simulink model "testing"  (R2025b)
settings: Solver=VariableStepAuto  StartTime=0.0  StopTime=50  RelTol=1e-3
values from neighbouring files (symbols this model uses):
  Area = 2*L*Width    (= 0.072)    [quad_params.m]
  end_h = 0.03    [quad_params.m]
  g = 9.81    [quad_params.m]
  h = [0 ... (first row only)    [Madgwick.m]    (also in quad_params.m = 0.2; umich_learning.m = x(:,1))
  h0 = Ts    (= 0.001)    [quad_params.m]
  inertia_mx = [Ixx; Iyy; Izz;]    [quad_params.m]
  init_h = 0.03    [quad_params.m]
  K_alloc = Alloc \ diag([W, 1, 1, 1])    [quad_params.m]
  r0_angle = 1000    [quad_params.m]
  r0_position = 1    [quad_params.m]
  rho_air = 1.225    [quad_params.m]
  rho_water = 1000    [quad_params.m]
  Trot = 0.01    [quad_params.m]
  Ts = 0.001    [get_noise.m]    (also in quad_params.m; test.m = 0.002)
  W = 0.7 + 4*m_prop    (= 0.74)    [quad_params.m]
undefined symbols (not defined in the file or in its folder): Alloc_2, b0, b0_pitch, b0_roll, b0_x, b0_y, b0_yaw, b0_z, beta1_pitch, beta1_roll, beta1_x, beta1_y, beta1_yaw, beta1_z, beta2_pitch, beta2_roll, beta2_x, beta2_y, beta2_yaw, beta2_z, beta3_pitch, beta3_roll, beta3_x, beta3_y, beta3_yaw, beta3_z, m, wc, wc_pitch, wc_roll, wc_x, wc_y, wc_yaw, wc_z, wo
libraries: simulink x3, shareduavrstlib x2, SignalEditorBlockLib x2, aerolibwind2 x1
(part 1 of 2)
settings Model: Creator=David  LastModifiedBy=David

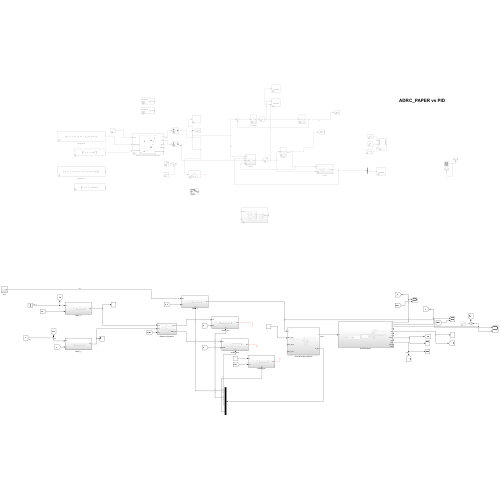
[thumbnail: Simulink's stored preview of the top-level diagram]
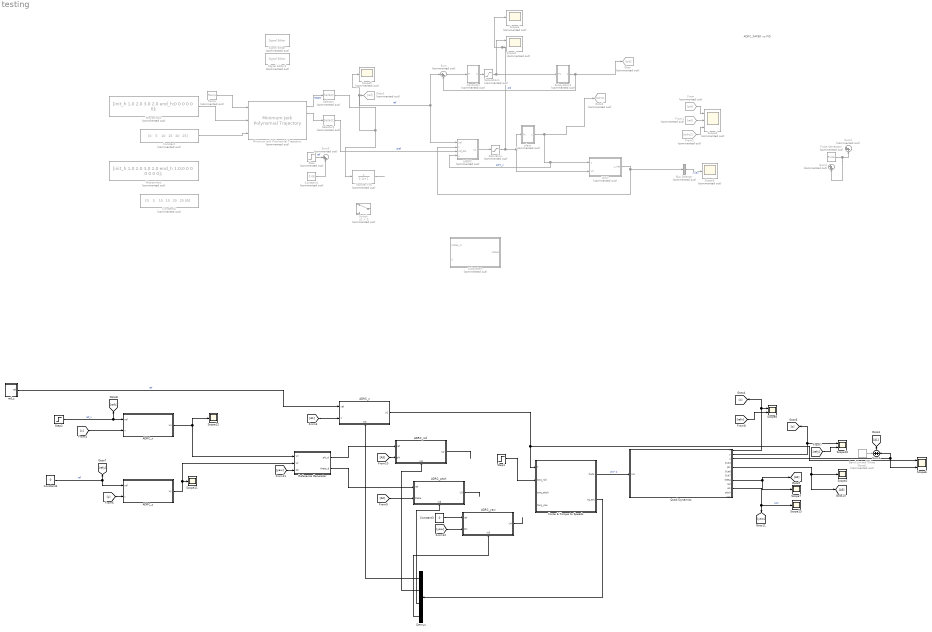
== system testing ==
  note: ADRC_PAPER vs PID
  ADRC_pitch : Subsystem
      settings: PortSchema="{\"entries\":[{\"content\":{\"sides\":[{\"content\":{\"connectorIds\":[\"In1\",\"In2\"]},\"type\":\"ConnectorPlacement.EquallySpacedRectSide\",\"uuid\":\"6cc80560-d5fb-4d70-bab2-c51ed037dc75\"},{\"content\":{\"connectorIds\":[\"Out1\"],\"side\":\"RIGHT\"},\"type\":\"ConnectorPlacement.EquallySpacedRectSide\",\"uuid\":\"11bda7cd-3ac7-47c0-848b-d0ab204a3c3d\"},{\"content\":{\"side\":\"TOP\"},\"type\":\"ConnectorPlacement.EquallySpacedRectSide\",\"uuid\":\"2a4fd4ae-6a0e-48eb-9f11-b11d2041070f\"},{\"content\":{\"connectorIds\":[\"In3\"],\"side\":\"BOTTOM\"},\"type\":\"ConnectorPlacement.EquallySpacedRectSide\",\"uuid\":\"f4a2dede-c3a4-45a0-96a3-5f68fdbf4ab0\"}]},\"type\":\"ConnectorPlacement.EquallySpacedConnector\",\"uuid\":\"bf44a222-f2d1-4d7f-8b8f-a2aef4aa21c8\"}],\"packageUris\":[\"http://schema.mathworks.com/mf0/Connector/R2020b\"],\"version\":\"1.0\"}"
  ADRC_roll : Subsystem
      settings: PortSchema="{\"entries\":[{\"content\":{\"sides\":[{\"content\":{\"connectorIds\":[\"In1\",\"In2\"]},\"type\":\"ConnectorPlacement.EquallySpacedRectSide\",\"uuid\":\"6cc80560-d5fb-4d70-bab2-c51ed037dc75\"},{\"content\":{\"connectorIds\":[\"Out1\"],\"side\":\"RIGHT\"},\"type\":\"ConnectorPlacement.EquallySpacedRectSide\",\"uuid\":\"11bda7cd-3ac7-47c0-848b-d0ab204a3c3d\"},{\"content\":{\"side\":\"TOP\"},\"type\":\"ConnectorPlacement.EquallySpacedRectSide\",\"uuid\":\"2a4fd4ae-6a0e-48eb-9f11-b11d2041070f\"},{\"content\":{\"connectorIds\":[\"In3\"],\"side\":\"BOTTOM\"},\"type\":\"ConnectorPlacement.EquallySpacedRectSide\",\"uuid\":\"852e14b7-d2e0-4511-9e4e-b55cc1d4afdd\"}]},\"type\":\"ConnectorPlacement.EquallySpacedConnector\",\"uuid\":\"bf44a222-f2d1-4d7f-8b8f-a2aef4aa21c8\"}],\"packageUris\":[\"http://schema.mathworks.com/mf0/Connector/R2020b\"],\"version\":\"1.0\"}"
  ADRC_x : Subsystem
  ADRC_y : Subsystem
  ADRC_yaw : Subsystem
      settings: PortSchema="{\"entries\":[{\"content\":{\"sides\":[{\"content\":{\"connectorIds\":[\"In1\",\"In2\"]},\"type\":\"ConnectorPlacement.EquallySpacedRectSide\",\"uuid\":\"6cc80560-d5fb-4d70-bab2-c51ed037dc75\"},{\"content\":{\"connectorIds\":[\"Out1\"],\"side\":\"RIGHT\"},\"type\":\"ConnectorPlacement.EquallySpacedRectSide\",\"uuid\":\"11bda7cd-3ac7-47c0-848b-d0ab204a3c3d\"},{\"content\":{\"side\":\"TOP\"},\"type\":\"ConnectorPlacement.EquallySpacedRectSide\",\"uuid\":\"2a4fd4ae-6a0e-48eb-9f11-b11d2041070f\"},{\"content\":{\"connectorIds\":[\"In3\"],\"side\":\"BOTTOM\"},\"type\":\"ConnectorPlacement.EquallySpacedRectSide\",\"uuid\":\"76ba5801-5866-4633-be25-22afc3afb05e\"}]},\"type\":\"ConnectorPlacement.EquallySpacedConnector\",\"uuid\":\"bf44a222-f2d1-4d7f-8b8f-a2aef4aa21c8\"}],\"packageUris\":[\"http://schema.mathworks.com/mf0/Connector/R2020b\"],\"version\":\"1.0\"}"
  ADRC_z : Subsystem
      settings: PortSchema="{\"entries\":[{\"content\":{\"sides\":[{\"content\":{\"connectorIds\":[\"In1\",\"In2\"]},\"type\":\"ConnectorPlacement.EquallySpacedRectSide\",\"uuid\":\"6cc80560-d5fb-4d70-bab2-c51ed037dc75\"},{\"content\":{\"connectorIds\":[\"Out1\"],\"side\":\"RIGHT\"},\"type\":\"ConnectorPlacement.EquallySpacedRectSide\",\"uuid\":\"11bda7cd-3ac7-47c0-848b-d0ab204a3c3d\"},{\"content\":{\"side\":\"TOP\"},\"type\":\"ConnectorPlacement.EquallySpacedRectSide\",\"uuid\":\"2a4fd4ae-6a0e-48eb-9f11-b11d2041070f\"},{\"content\":{\"connectorIds\":[\"In3\"],\"side\":\"BOTTOM\"},\"type\":\"ConnectorPlacement.EquallySpacedRectSide\",\"uuid\":\"eaf2a28a-e13e-4347-87b8-9ecab679d798\"}]},\"type\":\"ConnectorPlacement.EquallySpacedConnector\",\"uuid\":\"bf44a222-f2d1-4d7f-8b8f-a2aef4aa21c8\"}],\"packageUris\":[\"http://schema.mathworks.com/mf0/Connector/R2020b\"],\"version\":\"1.0\"}"
  Band-Limited White Noise1 : simulink/Sources/Band-Limited White Noise  Commented=on  Cov=[2.5*10^-9]  Ts=Ts  seed=[23341]
  Bus Selector : BusSelector  Commented=on  OutputSignals=x3
  Constant : Constant  Commented=on  Value="[0    5    10   15   20   25]"
  Constant1 : Constant  Commented=on  Value=0.06
  Constant2 : Constant  Commented=on  Value="[0    5    10   15   20   25 30]"
  Constant3 : Constant  Value=0
  Constant4 : Constant  Value=0
  Controller : Subsystem  Commented=on
  Demux : Demux
  Force & Torque to Speeds : Subsystem
  From : From  Commented=on  GotoTag=pid
  From1 : From  Commented=on  GotoTag=ref
  From2 : From  Commented=on  GotoTag=adrc2
  Goto : Goto  Commented=on  GotoTag=pid
  Goto1 : Goto  Commented=on  GotoTag=ref
  Goto2 : Goto  Commented=on  GotoTag=adrc2
  LADRC : Subsystem  Commented=on
  LESO : Subsystem  Commented=on
  Minimum Jerk Polynomial Trajectory : shareduavrstlib/Minimum Jerk Polynomial Trajectory  Commented=on  ShowBCInputPort=off  ShowPolynomialCoefs=off  ShowStatusOutputPort=off  TimeAllocation=off  TimeWeight=100  MinSegmentTime=0.1  MaxSegmentTime=1  MaxIteration=1500  MaxTime=10  SimulateUsing=Interpreted execution
  Pulse Generator : DiscretePulseGenerator  Commented=on  PulseType=Time based  Amplitude=0  Period=10  PulseWidth=5  PhaseDelay=5
  Quad Dynamics : Subsystem
  Ramp : simulink/Sources/Ramp  Commented=on  slope=1  start=0  InitialOutput=0
  Reference Generator : Subsystem
  Saturation : Saturate  Commented=on  UpperLimit=20  LowerLimit=0
  Saturation1 : Saturate  Commented=on  UpperLimit=20  LowerLimit=0
  Scope1 : Scope  Commented=on  NumInputPorts=2
      settings: ActiveDisplayYMinimum=-2.4999999999999996  ActiveDisplayYMaximum=22.5  DataLoggingVariableName=ScopeData3
  Scope10 : Scope  NumInputPorts=2
      settings: ActiveDisplayYMinimum=-0.76382760125435889  ActiveDisplayYMaximum=0.084869733472706529  DataLoggingVariableName=ScopeData16
  Scope{2,7,11..13} (5 alike) : Scope
      Scope11 settings: ActiveDisplayYMinimum=-170297.25681177425  ActiveDisplayYMaximum=18963.170251477775  DataLoggingVariableName=ScopeData17
      Scope12 settings: ActiveDisplayYMinimum=-1  ActiveDisplayYMaximum=1  DataLoggingVariableName=ScopeData13
      Scope13 settings: ActiveDisplayYMinimum=-0.0062641916569496255  ActiveDisplayYMaximum=0.056377724912546646  DataLoggingVariableName=ScopeData15
      Scope2 settings: ActiveDisplayYMinimum=-0.037678407203336144  ActiveDisplayYMaximum=0.035672125055144124  DataLoggingVariableName=ScopeData18
      Scope7 settings: ActiveDisplayYMinimum=-1  ActiveDisplayYMaximum=1  DataLoggingVariableName=ScopeData20
  Scope3 : Scope  Commented=on  NumInputPorts=3
      settings: ActiveDisplayYMinimum=-0.39386091056351047  ActiveDisplayYMaximum=3.5447481950715951  DataLoggingVariableName=ScopeData6
  Scope4 : Scope  Commented=on
      settings: ActiveDisplayYMinimum=-2.4999999999999996  ActiveDisplayYMaximum=22.5  DataLoggingVariableName=ScopeData5
  Scope5 : Scope  Commented=on
      settings: ActiveDisplayYMinimum=-236.47589926430294  ActiveDisplayYMaximum=517.92402381038687  DataLoggingVariableName=ScopeData7
  Scope6 : Scope  NumInputPorts=2
      settings: ActiveDisplayYMinimum=-7.7648917417809615  ActiveDisplayYMaximum=22.539500513991037  DataLoggingVariableName=ScopeData19
  Scope8 : Scope  NumInputPorts=2
      settings: ActiveDisplayYMinimum=-0.57257769005071735  ActiveDisplayYMaximum=0.3969530766723019  DataLoggingVariableName=ScopeData23
  Scope9 : Scope  Commented=on
      settings: ActiveDisplayYMinimum=-0.27915282069120229  ActiveDisplayYMaximum=3.5123753862208211  DataLoggingVariableName=ScopeData12
  Selector : Selector  Commented=on  InputPortWidth=2  IndexOptions=Index vector (dialog)  Indices=1  OutputSizes=1
  Selector1 : Selector  Commented=on  InputPortWidth=2  IndexOptions=Index vector (dialog)  Indices=1  OutputSizes=1
  Signal Editor : SignalEditorBlockLib/Signal Editor  Commented=on  FileName=untitled.mat  ActiveScenario=Scenario  ActiveSignal=Signal 1  IsBus=off  OutputBusObjectStr=Bus: BusObject  SampleTime=0  ZeroCross=off  OutputAfterFinalValue=Setting to zero  Unit=inherit  PreserveSignalName=on  ApplySigPropsToAllScenarios=on  ApplySigPropsToAllSignals=off  SignalPropertySource=Dialog parameters
  Signal Editor1 : SignalEditorBlockLib/Signal Editor  Commented=on  FileName=ref2.mat  ActiveScenario=Scenario  ActiveSignal=Signal2  IsBus=off  OutputBusObjectStr=Bus: BusObject  SampleTime=0  ZeroCross=off  OutputAfterFinalValue=Setting to zero  Unit=inherit  PreserveSignalName=on  ApplySigPropsToAllScenarios=on  ApplySigPropsToAllSignals=off  SignalPropertySource=Dialog parameters
  Step : Step  Commented=on  SampleTime=0
  Step1 : Step  Time=10  After=10  SampleTime=0
  Step2 : Step  Time=5  After=0.3  SampleTime=Ts
  Subsystem : Subsystem  Commented=on
  Subsystem3 : Subsystem  Commented=on
  Sum : Sum  Commented=on  Inputs=|+-
  Sum1 : Sum  Commented=on  Inputs=|++
  Sum2 : Sum  Commented=on  Inputs=|++
  Sum3 : Sum  Commented=on  Inputs=|++
  Sum4 : Sum
  Switch : Switch  Commented=on  Criteria=u2 > Threshold  SaturateOnIntegerOverflow=off  InputSameDT=off
  Transfer Fcn : TransferFcn  Commented=on  Numerator=[1 0]  Denominator=[0.1 1]
  Waypoints1 : Constant  Commented=on  Value="[init_h  1.0  2.0  3.0  2.0  end_h 1.0;0 0 0 0 0 0 0];"
  Waypoints2 : Constant  Commented=on  Value="[init_h  1.0  2.0  3.0  2.0  end_h;0 0 0 0 0 0];"
  plant : Subsystem  Commented=on
  ref_z : Subsystem
  wires:
  Sum/1 -> Controller/1(E)
  Controller/1(U) -> Saturation1/1
  LESO/1(z_hat) -> LADRC/2(x), Bus Selector/1
  LADRC/1(U1) -> Saturation/1
  Waypoints2/1 -> Minimum Jerk Polynomial Trajectory/2
  Constant/1 -> Minimum Jerk Polynomial Trajectory/3
  Minimum Jerk Polynomial Trajectory/1 -> Selector/1  "height"
  Ramp/1 -> Minimum Jerk Polynomial Trajectory/1
  Minimum Jerk Polynomial Trajectory/2 -> Selector1/1
  Selector/1 -> Transfer Fcn/1, LADRC/1(ref), Sum/1, Scope9/1, Goto1/1  "ref"
  Selector1/1 -> LADRC/3(ref_dot)  "dref"
  Saturation/1 -> Scope4/1, Scope1/2, plant/1(Fu), LESO/2(U1)
  Saturation1/1 -> Subsystem3/1(Fu), Scope1/1
  plant/1(z) -> LADRC/4(z), LESO/1(z), Goto2/1  "adrc_z"
  Subsystem3/1(z) -> Goto/1, Sum/2  "pid"
  Bus Selector/1 -> Scope5/1  "<x3>"
  From/1 -> Scope3/1
  From1/1 -> Scope3/2
  From2/1 -> Scope3/3
  Transfer Fcn/1 -> ?
  Step/1 -> Sum3/1  "ref"
  Constant1/1 -> Sum3/2
  Pulse Generator/1 -> Sum1/2, Sum2/2
  ref_z/1(ref) -> ADRC_z/1(ref)  "ref"
  Step2/1 -> [refx], ADRC_x/1(ref)  "ref_x"
  Demux/1 -> ADRC_z/3(In3)
  Sum4/1 -> [A1]
  ADRC_y/1(Uy) -> Reference Generator/2(Uy), Scope11/1
  Constant4/1 -> ADRC_y/1(ref), [refy]  "ref"
  [refx] -> Scope8/2
  [A3] -> ADRC_roll/2(phi)
  Reference Generator/2(theta_d) -> ADRC_pitch/1(ref)
  Force & Torque to Speeds/2(tq_act) -> Demux/1
  ADRC_x/1(Ux) -> Scope12/1, Reference Generator/1(Ux)
  [A1] -> ADRC_z/2(z)
  Band-Limited White Noise1/1 -> Sum4/1
  [y] -> ADRC_y/2(y)
  ADRC_yaw/1(U4) -> ?
  Quad Dynamics/2(y) -> Scope10/1, [y]
  [x] -> ADRC_x/2(x)
  [A2] -> ADRC_pitch/2(theta)
  Quad Dynamics/1(x) -> Scope8/1, [x]
  Reference Generator/1(phi_d) -> ADRC_roll/1(ref)
  Demux/4 -> ADRC_yaw/3(In3)
  [yaw] -> ADRC_yaw/2(psi)
  Force & Torque to Speeds/1(Out1) -> Quad Dynamics/1(In1)  "Wd^2"
  [yaw] -> Reference Generator/3(psi)
  Quad Dynamics/5(phi) -> [A3], Scope2/1
  Constant3/1 -> ADRC_yaw/1(ref)
  Demux/3 -> ADRC_pitch/3(In3)
  Quad Dynamics/3(z) -> Scope6/2, Sum4/2
  Quad Dynamics/8(theta) -> [A2], Scope7/1
  Quad Dynamics/10(psi) -> [yaw], Scope13/1  "yaw"
  [refy] -> Scope10/2
  ADRC_roll/1(U2) -> ?
  ADRC_pitch/1(U3) -> ?
  Demux/2 -> ADRC_roll/3(In3)
  ADRC_z/1(U1) -> Force & Torque to Speeds/1(T), Scope6/1
  Step1/1 -> Force & Torque to Speeds/2(torq_roll)

== system testing/ADRC_pitch ==
  ref : Inport
  theta : Inport  Port=2
  In3 : Inport  Port=3
  Bus Selector1 : BusSelector  Commented=on  OutputSignals=x3,x1
  LADRC : Subsystem
  LESO : Subsystem
  Scope : Scope  NumInputPorts=2
      settings: ActiveDisplayYMinimum=-0.038425071268255763  ActiveDisplayYMaximum=0.0634086481671494  DataLoggingVariableName=ScopeData3
  Scope1 : Scope  NumInputPorts=2
      settings: ActiveDisplayYMinimum=-0.038425071268255763  ActiveDisplayYMaximum=0.0634086481671494  DataLoggingVariableName=ScopeData9
  Scope6 : Scope  Commented=on
      settings: ActiveDisplayYMinimum=-1.7735639903680922  ActiveDisplayYMaximum=2.4901305931130953  DataLoggingVariableName=ScopeData11
  Scope7 : Scope  Commented=on  NumInputPorts=2
      settings: ActiveDisplayYMinimum=-10.826635982413356  ActiveDisplayYMaximum=4.5963077407770285  DataLoggingVariableName=ScopeData7
  TD1 : Subsystem
  Transfer Fcn : TransferFcn  Commented=on  Denominator=[0.8 1]
  U3 : Outport
  wires:
  Transfer Fcn/1 -> Scope7/2
  TD1/1(ref) -> Scope/1, LADRC/1(ref)
  LESO/1(z_hat) -> LADRC/2(x_hat), Bus Selector1/1
  theta/1 -> LESO/1(theta)
  Bus Selector1/1 -> Transfer Fcn/1, Scope7/1  "<x3>"
  Bus Selector1/2 -> Scope6/1  "<x1>"
  LADRC/1(U3) -> Scope1/2, U3/1
  TD1/2(dref) -> LADRC/3(ref_dot)
  ref/1 -> TD1/1(v), Scope/2
  In3/1 -> Scope1/1, LESO/2(U3)

== system testing/ADRC_roll ==
  ref : Inport
  phi : Inport  Port=2
  In3 : Inport  Port=3
  Bus Selector1 : BusSelector  Commented=on  OutputSignals=x3,x1
  LADRC1 : Subsystem
  LESO1 : Subsystem
  Scope : Scope  NumInputPorts=2
      settings: ActiveDisplayYMinimum=-0.060213513903969583  ActiveDisplayYMaximum=0.059112792343212317  DataLoggingVariableName=ScopeData25
  Scope1 : Scope  NumInputPorts=2
      settings: ActiveDisplayYMinimum=-0.014376092531118703  ActiveDisplayYMaximum=0.015183833105855788  DataLoggingVariableName=ScopeData14
  Scope6 : Scope  Commented=on
      settings: ActiveDisplayYMinimum=-1.7735639903680922  ActiveDisplayYMaximum=2.4901305931130953  DataLoggingVariableName=ScopeData11
  Scope7 : Scope  Commented=on  NumInputPorts=2
      settings: ActiveDisplayYMinimum=-10.826635982413356  ActiveDisplayYMaximum=4.5963077407770285  DataLoggingVariableName=ScopeData7
  TD1 : Subsystem
  Transfer Fcn : TransferFcn  Commented=on  Denominator=[0.8 1]
  U2 : Outport
  wires:
  Bus Selector1/2 -> Scope6/1  "<x1>"
  Bus Selector1/1 -> Scope7/1, Transfer Fcn/1  "<x3>"
  phi/1 -> LESO1/1(phi)
  LESO1/1(z_hat) -> LADRC1/2(x_hat)
  Transfer Fcn/1 -> Scope7/2
  TD1/2(dref) -> LADRC1/3(ref_dot)
  TD1/1(ref) -> Scope/1, LADRC1/1(ref)
  LADRC1/1(U2) -> Scope1/2, U2/1
  ref/1 -> Scope/2, TD1/1(v)
  In3/1 -> Scope1/1, LESO1/2(U2)

== system testing/ADRC_x ==
  ref : Inport
  x : Inport  Port=2
  Bus Selector1 : BusSelector  Commented=on  OutputSignals=x3,x1
  LADRC1 : Subsystem
  LESO1 : Subsystem
  Scope : Scope  NumInputPorts=2
      settings: ActiveDisplayYMinimum=-0.027979577978769543  ActiveDisplayYMaximum=0.35850174610360214  DataLoggingVariableName=ScopeData3
  Scope6 : Scope  Commented=on
      settings: ActiveDisplayYMinimum=-1.7735639903680922  ActiveDisplayYMaximum=2.4901305931130953  DataLoggingVariableName=ScopeData11
  Scope7 : Scope  Commented=on  NumInputPorts=2
      settings: ActiveDisplayYMinimum=-10.826635982413356  ActiveDisplayYMaximum=4.5963077407770285  DataLoggingVariableName=ScopeData7
  TD1 : Subsystem
  Transfer Fcn : TransferFcn  Commented=on  Denominator=[0.8 1]
  Ux : Outport
  wires:
  ref/1 -> TD1/1(v), Scope/2
  TD1/2(dref) -> LADRC1/3(ref_dot)
  Bus Selector1/2 -> Scope6/1  "<x1>"
  Bus Selector1/1 -> Scope7/1, Transfer Fcn/1  "<x3>"
  x/1 -> LESO1/1(x)
  LESO1/1(z_hat) -> Bus Selector1/1, LADRC1/2(x_hat)
  TD1/1(ref) -> LADRC1/1(ref), Scope/1
  Transfer Fcn/1 -> Scope7/2
  LADRC1/1(U1) -> Ux/1, LESO1/2(U1)

== system testing/ADRC_y ==
  ref : Inport
  y : Inport  Port=2
  Bus Selector1 : BusSelector  Commented=on  OutputSignals=x3,x1
  LADRC1 : Subsystem
  LESO1 : Subsystem
  Scope6 : Scope  Commented=on
      settings: ActiveDisplayYMinimum=-4.0118283317897359E-5  ActiveDisplayYMaximum=0.00036106454986107629  DataLoggingVariableName=ScopeData11
  Scope7 : Scope  Commented=on  NumInputPorts=2
      settings: ActiveDisplayYMinimum=-42.604143461795488  ActiveDisplayYMaximum=4.7337937179772753  DataLoggingVariableName=ScopeData7
  TD1 : Subsystem
  Transfer Fcn : TransferFcn  Commented=on  Denominator=[0.8 1]
  Uy : Outport
  wires:
  Transfer Fcn/1 -> Scope7/2
  TD1/1(ref) -> LADRC1/1(ref)
  LESO1/1(y_hat) -> LADRC1/2(y_hat)
  y/1 -> LESO1/1(y)
  Bus Selector1/1 -> Transfer Fcn/1, Scope7/1  "<x3>"
  Bus Selector1/2 -> Scope6/1  "<x1>"
  TD1/2(dref) -> LADRC1/3(ref_dot)
  ref/1 -> TD1/1(v)
  LADRC1/1(U1) -> LESO1/2(U1), Uy/1

== system testing/ADRC_yaw ==
  ref : Inport
  psi : Inport  Port=2
  In3 : Inport  Port=3
  Bus Selector1 : BusSelector  Commented=on  OutputSignals=x3,x1
  LADRC1 : Subsystem
  LESO1 : Subsystem
  Scope : Scope  NumInputPorts=2
      settings: ActiveDisplayYMinimum=-0.0062687034065030244  ActiveDisplayYMaximum=0.056418330658527235  DataLoggingVariableName=ScopeData3
  Scope6 : Scope  Commented=on
      settings: ActiveDisplayYMinimum=-1.7735639903680922  ActiveDisplayYMaximum=2.4901305931130953  DataLoggingVariableName=ScopeData11
  Scope7 : Scope  Commented=on  NumInputPorts=2
      settings: ActiveDisplayYMinimum=-10.826635982413356  ActiveDisplayYMaximum=4.5963077407770285  DataLoggingVariableName=ScopeData7
  TD1 : Subsystem
  Transfer Fcn : TransferFcn  Commented=on  Denominator=[0.8 1]
  U4 : Outport
  wires:
  Transfer Fcn/1 -> Scope7/2
  TD1/1(ref) -> Scope/1, LADRC1/1(ref)
  LESO1/1(z_hat) -> LADRC1/2(x_hat), Bus Selector1/1
  psi/1 -> LESO1/1(theta)
  Bus Selector1/1 -> Transfer Fcn/1, Scope7/1  "<x3>"
  Bus Selector1/2 -> Scope6/1  "<x1>"
  TD1/2(dref) -> LADRC1/3(ref_dot)
  ref/1 -> TD1/1(v), Scope/2
  LADRC1/1(U1) -> U4/1
  In3/1 -> LESO1/2(U1)

== system testing/ADRC_z ==
  ref : Inport
  z : Inport  Port=2
  In3 : Inport  Port=3
  Bus Selector1 : BusSelector  Commented=on  OutputSignals=x3,x1
  Gain1 : Gain  Commented=through  Gain=W
  Gain2 : Gain  Commented=through  Gain=1/W
  LADRC1 : Subsystem
  LESO1 : Subsystem
  Scope : Scope  NumInputPorts=2
      settings: ActiveDisplayYMinimum=-1  ActiveDisplayYMaximum=1  DataLoggingVariableName=ScopeData3
  Scope6 : Scope  Commented=on
      settings: ActiveDisplayYMinimum=-1.7735639903680922  ActiveDisplayYMaximum=2.4901305931130953  DataLoggingVariableName=ScopeData11
  Scope7 : Scope  Commented=on  NumInputPorts=2
      settings: ActiveDisplayYMinimum=-10.826635982413356  ActiveDisplayYMaximum=4.5963077407770285  DataLoggingVariableName=ScopeData7
  TD1 : Subsystem
  Transfer Fcn : TransferFcn  Commented=on  Denominator=[0.8 1]
  U1 : Outport
  wires:
  ref/1 -> Scope/2, TD1/1(v)
  TD1/2(dref) -> LADRC1/3(ref_dot)
  LADRC1/1(U1) -> Gain1/1
  Bus Selector1/2 -> Scope6/1  "<x1>"
  Bus Selector1/1 -> Scope7/1, Transfer Fcn/1  "<x3>"
  z/1 -> LESO1/1(z)
  LESO1/1(z_hat) -> Bus Selector1/1, LADRC1/2(x_hat)
  TD1/1(ref) -> Scope/1, LADRC1/1(ref)
  Transfer Fcn/1 -> Scope7/2
  Gain1/1 -> U1/1
  In3/1 -> Gain2/1
  Gain2/1 -> LESO1/2(U1)

== system testing/Controller ==
  E : Inport
  Derivative : Derivative
  Gain : Gain  Gain=25
  Gain1 : Gain  Gain=3
  Gain2 : Gain  Gain=10
  Integrator2 : Integrator
  Scope : Scope
      settings: ActiveDisplayYMinimum=-1  ActiveDisplayYMaximum=1
  Scope1 : Scope
      settings: ActiveDisplayYMinimum=-1  ActiveDisplayYMaximum=1
  Sum3 : Sum  Inputs=|+++
  U : Outport
  wires:
  Gain/1 -> Scope1/1, Sum3/2
  E/1 -> Gain/1, Gain1/1, Gain2/1
  Derivative/1 -> Sum3/3
  Gain1/1 -> Derivative/1
  Gain2/1 -> Integrator2/1
  Integrator2/1 -> Scope/1, Sum3/1
  Sum3/1 -> U/1

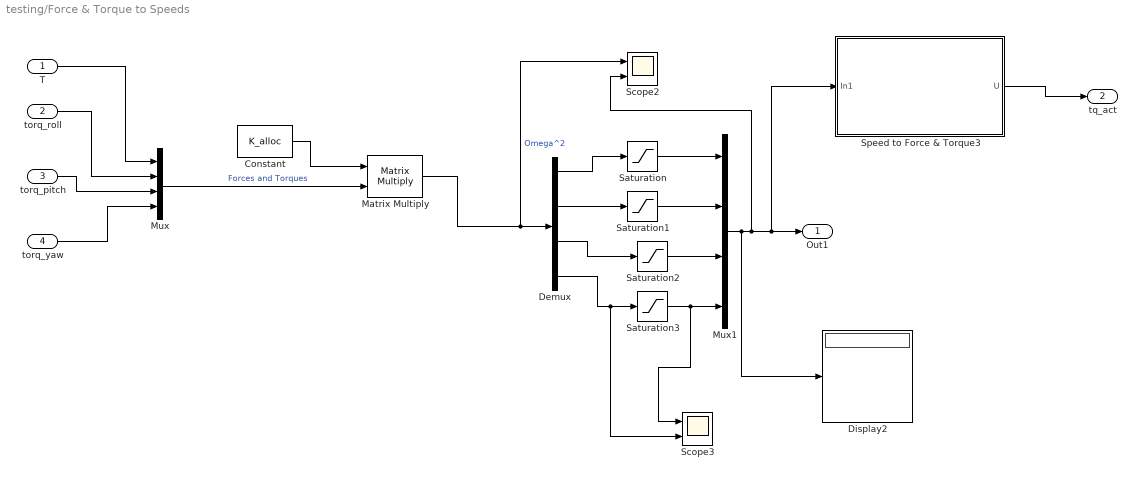
== system testing/Force & Torque to Speeds ==
  T : Inport
  torq_roll : Inport  Port=2
  torq_pitch : Inport  Port=3
  torq_yaw : Inport  Port=4
  Constant : Constant  Value=K_alloc
  Demux : Demux
  Display2 : Display
  Matrix Multiply : Product  Multiplication=Matrix(*)
  Mux : Mux
  Mux1 : Mux
  Saturation{,1..3} (4 alike) : Saturate  UpperLimit=10^10  LowerLimit=0
  Scope2 : Scope  NumInputPorts=2
      settings: ActiveDisplayYMinimum=-267783.50137100497  ActiveDisplayYMaximum=199309.4437307195  DataLoggingVariableName=ScopeData21
  Scope3 : Scope  NumInputPorts=2
      settings: ActiveDisplayYMinimum=-45060.545766456409  ActiveDisplayYMaximum=35485.477502733229  DataLoggingVariableName=ScopeData21
  Speed to Force & Torque3 : Subsystem
  Out1 : Outport
  tq_act : Outport  Port=2
  wires:
  Matrix Multiply/1 -> Scope2/1, Demux/1  "Omega^2"
  torq_yaw/1 -> Mux/4
  torq_pitch/1 -> Mux/3
  torq_roll/1 -> Mux/2
  T/1 -> Mux/1
  Constant/1 -> Matrix Multiply/1
  Mux/1 -> Matrix Multiply/2  "Forces and Torques"
  Saturation3/1 -> Scope3/1, Mux1/4
  Demux/4 -> Scope3/2, Saturation3/1
  Demux/2 -> Saturation1/1
  Demux/1 -> Saturation/1
  Demux/3 -> Saturation2/1
  Saturation1/1 -> Mux1/2
  Saturation/1 -> Mux1/1
  Saturation2/1 -> Mux1/3
  Mux1/1 -> Display2/1, Scope2/2, Speed to Force & Torque3/1(In1), Out1/1
  Speed to Force & Torque3/1(U) -> tq_act/1

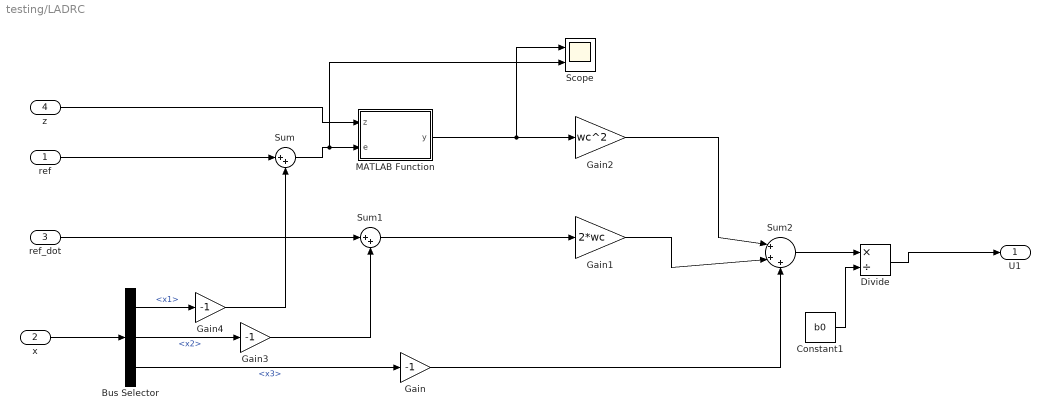
== system testing/LADRC ==
  ref : Inport
  x : Inport  Port=2
  ref_dot : Inport  Port=3
  z : Inport  Port=4
  Bus Selector : BusSelector  OutputSignals=x1,x2,x3
  Constant1 : Constant  Value=b0
  Divide : Product  Inputs=*/
  Gain : Gain  Gain=-1
  Gain1 : Gain  Gain=2*wc
  Gain2 : Gain  Gain=wc^2
  Gain3 : Gain  Gain=-1
  Gain4 : Gain  Gain=-1
  MATLAB Function : MATLAB Function  TreatAsAtomicUnit=on
  Scope : Scope  NumInputPorts=2
      settings: ActiveDisplayYMinimum=-0.091781366249220786  ActiveDisplayYMaximum=0.232420151805469  DataLoggingVariableName=ScopeData2
  Sum : Sum  Inputs=|++
  Sum1 : Sum  Inputs=|++
  Sum2 : Sum  Inputs=|+++
  U1 : Outport
  wires:
  Sum2/1 -> Divide/1
  x/1 -> Bus Selector/1
  Bus Selector/3 -> Gain/1  "<x3>"
  Gain2/1 -> Sum2/1
  Gain/1 -> Sum2/3
  Gain1/1 -> Sum2/2
  Bus Selector/1 -> Gain4/1  "<x1>"
  Bus Selector/2 -> Gain3/1  "<x2>"
  Gain4/1 -> Sum/2
  Gain3/1 -> Sum1/2
  ref_dot/1 -> Sum1/1
  Sum1/1 -> Gain1/1
  Divide/1 -> U1/1
  Constant1/1 -> Divide/2
  ref/1 -> Sum/1
  MATLAB Function/1(y) -> Scope/1, Gain2/1
  z/1 -> MATLAB Function/1(z)
  Sum/1 -> Scope/2, MATLAB Function/2(e)

== system testing/LESO ==
  z : Inport
  U1 : Inport  Port=2
  Bus Creator : BusCreator  Inputs=3
  Gain : Gain  Gain=-3*wo
  Gain1 : Gain  Gain=-1
  Gain2 : Gain  Gain=-3*(wo^2)
  Gain3 : Gain  Gain=-(wo^3)
  Gain4 : Gain  Gain=b0
  Integrator : Integrator
  Integrator1 : Integrator
  Integrator2 : Integrator
  Sum : Sum  Inputs=|++
  Sum1 : Sum  Inputs=|++
  Sum2 : Sum  Inputs=|+++
  z_hat : Outport
  wires:
  z/1 -> Gain1/1
  Gain1/1 -> Sum/1
  Sum/1 -> Gain3/1, Gain2/1, Gain/1
  Integrator/1 -> Sum/2, Bus Creator/1  "x1"
  Gain3/1 -> Integrator2/1  "x3_dot"
  Bus Creator/1 -> z_hat/1
  Sum1/1 -> Integrator/1  "x1_dot"
  Gain/1 -> Sum1/1
  Integrator1/1 -> Bus Creator/2, Sum1/2  "x2"
  Integrator2/1 -> Bus Creator/3, Sum2/2  "x3"
  Gain2/1 -> Sum2/1
  Sum2/1 -> Integrator1/1  "x2_dot"
  U1/1 -> Gain4/1
  Gain4/1 -> Sum2/3

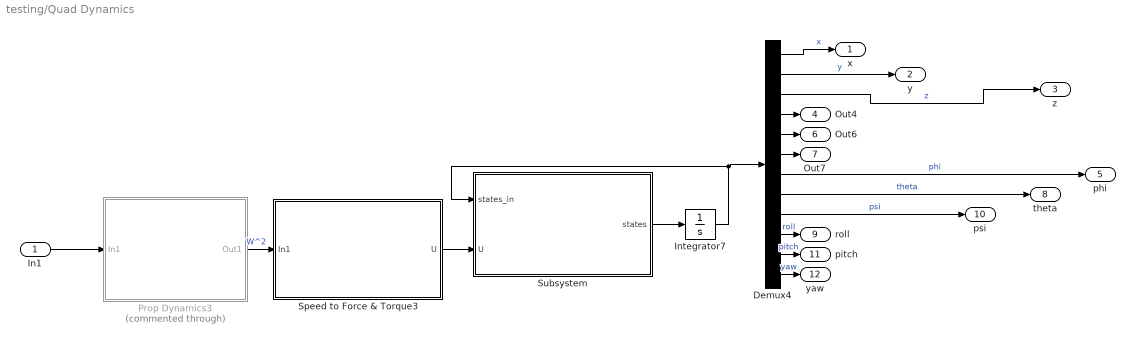
== system testing/Quad Dynamics ==
  In1 : Inport
  Demux4 : Demux  Outputs=12
  Integrator7 : Integrator  InitialCondition=zeros(12,1)
  Prop Dynamics3 : Subsystem  Commented=through
  Speed to Force & Torque3 : Subsystem
  Subsystem : Subsystem
  x : Outport
  y : Outport  Port=2
  z : Outport  Port=3
  Out4 : Outport  Port=4
  phi : Outport  Port=5
  Out6 : Outport  Port=6
  Out7 : Outport  Port=7
  theta : Outport  Port=8
  roll : Outport  Port=9
  psi : Outport  Port=10
  pitch : Outport  Port=11
  yaw : Outport  Port=12
  wires:
  Demux4/2 -> y/1  "y"
  Prop Dynamics3/1(Out1) -> Speed to Force & Torque3/1(In1)  "W^2"
  Demux4/1 -> x/1  "x"
  Subsystem/1(states) -> Integrator7/1
  Speed to Force & Torque3/1(U) -> Subsystem/2(U)
  Integrator7/1 -> Demux4/1, Subsystem/1(states_in)
  Demux4/10 -> roll/1  "roll"
  Demux4/7 -> phi/1  "phi"
  Demux4/3 -> z/1  "z"
  Demux4/9 -> psi/1  "psi"
  Demux4/8 -> theta/1  "theta"
  Demux4/11 -> pitch/1  "pitch"
  Demux4/12 -> yaw/1  "yaw"
  Demux4/6 -> Out7/1
  Demux4/5 -> Out6/1
  Demux4/4 -> Out4/1
  In1/1 -> Prop Dynamics3/1(In1)

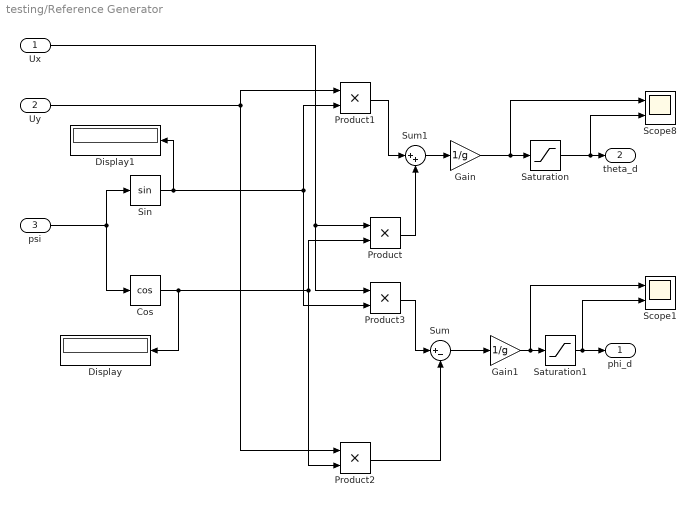
== system testing/Reference Generator ==
  Ux : Inport
  Uy : Inport  Port=2
  psi : Inport  Port=3
  Cos : Trigonometry  Operator=cos
  Display : Display
  Display1 : Display
  Gain : Gain  Gain=1/g
  Gain1 : Gain  Gain=1/g
  Product{,1..3} (4 alike) : Product
  Saturation : Saturate  UpperLimit=0.52  LowerLimit=-0.52
  Saturation1 : Saturate  UpperLimit=0.52  LowerLimit=-0.52
  Scope1 : Scope  NumInputPorts=2
      settings: ActiveDisplayYMinimum=-0.063445456668569211  ActiveDisplayYMaximum=0.070247465499666387  DataLoggingVariableName=ScopeData8
  Scope8 : Scope  NumInputPorts=2
      settings: ActiveDisplayYMinimum=-0.54055917517100971  ActiveDisplayYMaximum=0.39565615173394986  DataLoggingVariableName=ScopeData4
  Sin : Trigonometry
  Sum : Sum  Inputs=|+-
  Sum1 : Sum  Inputs=|++
  phi_d : Outport
  theta_d : Outport  Port=2
  wires:
  psi/1 -> Cos/1, Sin/1
  Cos/1 -> Display/1, Product2/2, Product/2
  Ux/1 -> Product3/1, Product/1
  Uy/1 -> Product2/1, Product1/1
  Product1/1 -> Sum1/1
  Product/1 -> Sum1/2
  Sum1/1 -> Gain/1
  Gain/1 -> Scope8/1, Saturation/1
  Product2/1 -> Sum/2
  Product3/1 -> Sum/1
  Sum/1 -> Gain1/1
  Gain1/1 -> Scope1/1, Saturation1/1
  Sin/1 -> Product3/2, Product1/2, Display1/1
  Saturation/1 -> Scope8/2, theta_d/1
  Saturation1/1 -> Scope1/2, phi_d/1

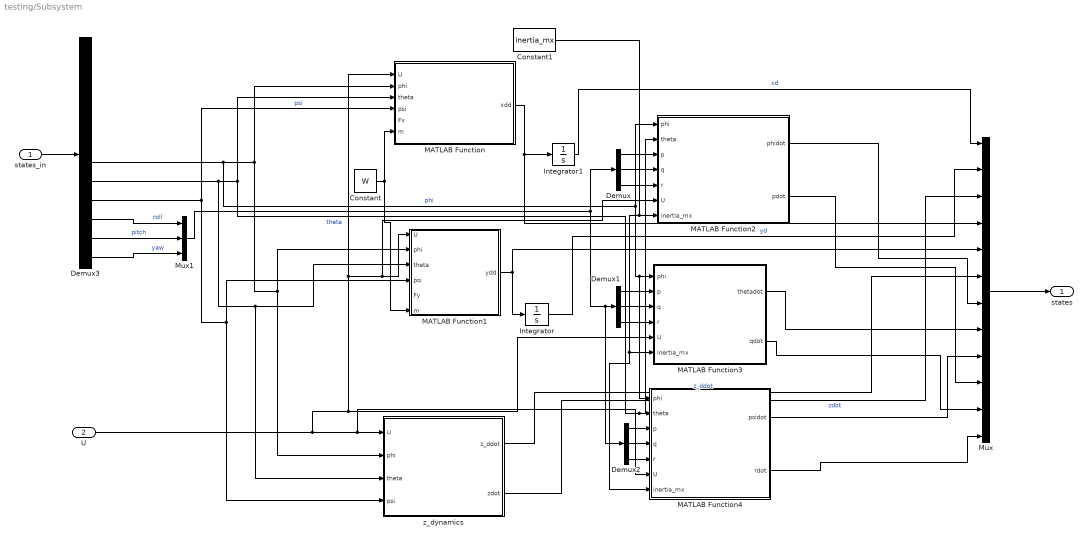
== system testing/Subsystem ==
  states_in : Inport
  U : Inport  Port=2
  Constant : Constant  Value=W
  Constant1 : Constant  Value=inertia_mx
  Demux : Demux  Outputs=3
  Demux1 : Demux  Outputs=3
  Demux2 : Demux  Outputs=3
  Demux3 : Demux  Outputs=12
  Integrator : Integrator
  Integrator1 : Integrator
  MATLAB Function : MATLAB Function  TreatAsAtomicUnit=on
  MATLAB Function1 : MATLAB Function  TreatAsAtomicUnit=on
  MATLAB Function2 : MATLAB Function  TreatAsAtomicUnit=on
  MATLAB Function3 : MATLAB Function  TreatAsAtomicUnit=on
  MATLAB Function4 : MATLAB Function  TreatAsAtomicUnit=on
  Mux : Mux  Inputs=12
  Mux1 : Mux  Inputs=3
  z_dynamics : Subsystem
  states : Outport
  wires:
  MATLAB Function/1(xdd) -> Mux/4, Integrator1/1
  MATLAB Function1/1(ydd) -> Integrator/1, Mux/5
  Integrator1/1 -> Mux/1  "xd"
  Integrator/1 -> Mux/2  "yd"
  z_dynamics/2(zdot) -> Mux/3  "zdot"
  z_dynamics/1(z_ddot) -> Mux/6  "z_ddot"
  MATLAB Function2/1(phidot) -> Mux/7
  MATLAB Function3/1(thetadot) -> Mux/8
  MATLAB Function4/1(psidot) -> Mux/9
  MATLAB Function2/2(pdot) -> Mux/10
  MATLAB Function3/2(qdot) -> Mux/11
  MATLAB Function4/2(rdot) -> Mux/12
  Mux/1 -> states/1
  states_in/1 -> Demux3/1
  U/1 -> MATLAB Function/1(U), MATLAB Function2/6(U), MATLAB Function1/1(U), MATLAB Function3/5(U), MATLAB Function4/6(U), z_dynamics/1(U)
  Demux3/7 -> MATLAB Function3/1(phi), MATLAB Function4/1(phi), MATLAB Function2/1(phi), MATLAB Function/2(phi), z_dynamics/2(phi), MATLAB Function1/2(phi)  "phi"
  Demux3/8 -> z_dynamics/3(theta), MATLAB Function1/3(theta), MATLAB Function2/2(theta), MATLAB Function4/2(theta), MATLAB Function/3(theta)  "theta"
  Demux3/9 -> z_dynamics/4(psi), MATLAB Function1/4(psi), MATLAB Function/4(psi)  "psi"
  Constant/1 -> MATLAB Function1/6(m), MATLAB Function/6(m)
  Constant1/1 -> MATLAB Function4/7(inertia_mx), MATLAB Function3/6(inertia_mx), MATLAB Function2/7(inertia_mx)
  Demux3/11 -> Mux1/2  "pitch"
  Demux3/12 -> Mux1/3  "yaw"
  Demux3/10 -> Mux1/1  "roll"
  Mux1/1 -> Demux/1, Demux2/1, Demux1/1
  Demux1/1 -> MATLAB Function3/2(p)
  Demux1/2 -> MATLAB Function3/3(q)
  Demux1/3 -> MATLAB Function3/4(r)
  Demux2/1 -> MATLAB Function4/3(p)
  Demux2/2 -> MATLAB Function4/4(q)
  Demux2/3 -> MATLAB Function4/5(r)
  Demux/1 -> MATLAB Function2/3(p)
  Demux/2 -> MATLAB Function2/4(q)
  Demux/3 -> MATLAB Function2/5(r)

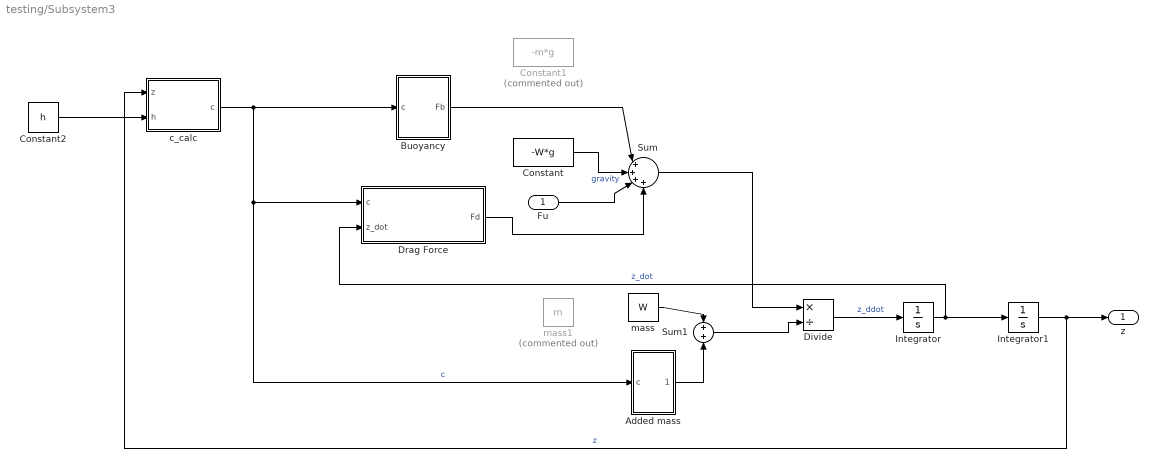
== system testing/Subsystem3 ==
  Fu : Inport
  Added mass : Subsystem
  Buoyancy : Subsystem
  Constant : Constant  Value=-W*g
  Constant1 : Constant  Commented=on  Value=-m*g
  Constant2 : Constant  Value=h
  Divide : Product  Inputs=*/
  Drag Force : Subsystem
  Integrator : Integrator
  Integrator1 : Integrator  InitialCondition=init_h
  Sum : Sum  Inputs=|++++
  Sum1 : Sum
  c_calc : MATLAB Function  TreatAsAtomicUnit=on
  mass : Constant  Value=W
  mass1 : Constant  Commented=on  Value=m
  z : Outport
  wires:
  Sum1/1 -> Divide/2
  mass/1 -> Sum1/1
  Integrator1/1 -> c_calc/1(z), z/1  "z"
  c_calc/1(c) -> Buoyancy/1(c), Added mass/1(c), Drag Force/1(c)  "c"
  Sum/1 -> Divide/1
  Integrator/1 -> Drag Force/2(z_dot), Integrator1/1  "z_dot"
  Divide/1 -> Integrator/1  "z_ddot"
  Fu/1 -> Sum/3
  Constant/1 -> Sum/2  "gravity"
  Constant2/1 -> c_calc/2(h)
  Drag Force/1(Fd) -> Sum/4
  Buoyancy/1(Fb) -> Sum/1
  Added mass/1(m_a) -> Sum1/2

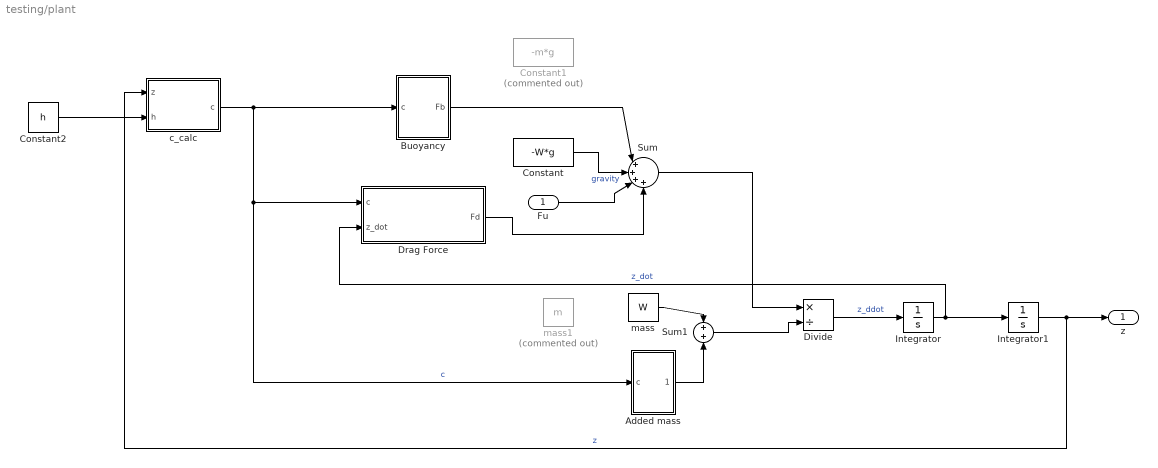
== system testing/plant ==
  Fu : Inport
  Added mass : Subsystem
  Buoyancy : Subsystem
  Constant : Constant  Value=-W*g
  Constant1 : Constant  Commented=on  Value=-m*g
  Constant2 : Constant  Value=h
  Divide : Product  Inputs=*/
  Drag Force : Subsystem
  Integrator : Integrator
  Integrator1 : Integrator  InitialCondition=init_h
  Sum : Sum  Inputs=|++++
  Sum1 : Sum
  c_calc : MATLAB Function  TreatAsAtomicUnit=on
  mass : Constant  Value=W
  mass1 : Constant  Commented=on  Value=m
  z : Outport
  wires:
  Added mass/1(m_a) -> Sum1/2
  Buoyancy/1(Fb) -> Sum/1
  Drag Force/1(Fd) -> Sum/4
  Constant2/1 -> c_calc/2(h)
  Constant/1 -> Sum/2  "gravity"
  Fu/1 -> Sum/3
  Divide/1 -> Integrator/1  "z_ddot"
  Integrator/1 -> Integrator1/1, Drag Force/2(z_dot)  "z_dot"
  Sum/1 -> Divide/1
  c_calc/1(c) -> Drag Force/1(c), Added mass/1(c), Buoyancy/1(c)  "c"
  Integrator1/1 -> z/1, c_calc/1(z)  "z"
  mass/1 -> Sum1/1
  Sum1/1 -> Divide/2

== system testing/ref_z ==
  Constant4 : Constant  Value=init_h
  Manual Switch4 : ManualSwitch  CurrentSetting=0
  Min Jerk Trajectory1 : Subsystem
  Step : Step  SampleTime=0
  Sum7 : Sum  Inputs=|++
  ref : Outport
  wires:
  Min Jerk Trajectory1/2(dref) -> ?
  Sum7/1 -> Manual Switch4/2  "v"
  Min Jerk Trajectory1/1(ref) -> Manual Switch4/1
  Constant4/1 -> Sum7/2
  Step/1 -> Sum7/1  "v"
  Manual Switch4/1 -> ref/1  "ref"

== system testing/ADRC_pitch/LADRC ==
  ref : Inport
  x_hat : Inport  Port=2
  ref_dot : Inport  Port=3
  Bus Selector1 : BusSelector  OutputSignals=x1,x2,x3
  Constant1 : Constant  Value=b0_pitch
  Divide : Product  Inputs=*/
  Gain5 : Gain  Gain=-1
  Gain6 : Gain  Gain=2*wc_pitch
  Gain7 : Gain  Gain=wc_pitch^2
  Gain8 : Gain  Gain=-1
  Gain9 : Gain  Gain=-1
  Sum3 : Sum  Inputs=|++
  Sum4 : Sum  Inputs=|++
  Sum5 : Sum  Inputs=|+++
  U3 : Outport
  wires:
  Gain7/1 -> Sum5/1
  Bus Selector1/2 -> Gain8/1  "<x2>"
  ref_dot/1 -> Sum4/1
  Gain6/1 -> Sum5/2
  Gain9/1 -> Sum3/2
  Gain8/1 -> Sum4/2
  Sum4/1 -> Gain6/1
  Sum3/1 -> Gain7/1
  Bus Selector1/1 -> Gain9/1  "<x1>"
  ref/1 -> Sum3/1
  Gain5/1 -> Sum5/3
  x_hat/1 -> Bus Selector1/1
  Divide/1 -> U3/1
  Bus Selector1/3 -> Gain5/1  "<x3>"
  Sum5/1 -> Divide/1
  Constant1/1 -> Divide/2

== system testing/ADRC_pitch/LESO ==
  theta : Inport
  U3 : Inport  Port=2
  Bus Creator : BusCreator  Inputs=3
  Gain : Gain  Gain=-beta1_pitch
  Gain1 : Gain  Gain=-1
  Gain2 : Gain  Gain=-beta2_pitch
  Gain3 : Gain  Gain=-beta3_pitch
  Gain4 : Gain  Gain=b0_pitch
  Integrator : Integrator
  Integrator1 : Integrator
  Integrator2 : Integrator
  Sum : Sum  Inputs=|++
  Sum1 : Sum  Inputs=|++
  Sum2 : Sum  Inputs=|+++
  z_hat : Outport
  wires:
  theta/1 -> Gain1/1
  Gain1/1 -> Sum/1
  Sum/1 -> Gain3/1, Gain2/1, Gain/1
  Integrator/1 -> Bus Creator/1, Sum/2  "x1"
  Gain3/1 -> Integrator2/1  "x3_dot"
  Bus Creator/1 -> z_hat/1
  Sum1/1 -> Integrator/1  "x1_dot"
  Gain/1 -> Sum1/1
  Integrator1/1 -> Bus Creator/2, Sum1/2  "x2"
  Integrator2/1 -> Bus Creator/3, Sum2/2  "x3"
  Gain2/1 -> Sum2/1
  Sum2/1 -> Integrator1/1  "x2_dot"
  U3/1 -> Gain4/1
  Gain4/1 -> Sum2/3

== system testing/ADRC_pitch/TD1 ==
  v : Inport
  Constant11 : Constant  Value=r0_angle
  Constant12 : Constant  Value=h0
  Delay One Step : Delay  DelayLength=1  SampleTime=Ts
  Delay One Step1 : Delay  DelayLength=1  SampleTime=Ts
  Gain3 : Gain  Gain=Ts
  Gain4 : Gain  Gain=Ts
  Sum1 : Sum  Inputs=|++
  Sum6 : Sum  Inputs=|++
  Sum7 : Sum  Inputs=|+-
  fhan : MATLAB Function  TreatAsAtomicUnit=on
  ref : Outport
  dref : Outport  Port=2
  wires:
  v/1 -> Sum7/2
  Gain3/1 -> Sum6/1
  Constant12/1 -> fhan/4(h0)
  Delay One Step/1 -> Sum1/1
  Gain4/1 -> Sum1/2
  Sum1/1 -> Sum7/1, Delay One Step/1, ref/1  "v1"
  Sum7/1 -> fhan/1(e)
  fhan/1(u) -> Gain3/1
  Sum6/1 -> Delay One Step1/1  "v2"
  Constant11/1 -> fhan/3(r0)
  Delay One Step1/1 -> Gain4/1, Sum6/2, fhan/2(v2), dref/1

== system testing/ADRC_roll/LADRC1 ==
  ref : Inport
  x_hat : Inport  Port=2
  ref_dot : Inport  Port=3
  Bus Selector : BusSelector  OutputSignals=x1,x2,x3
  Constant : Constant  Value=b0_roll
  Divide : Product  Inputs=*/
  Gain : Gain  Gain=-1
  Gain1 : Gain  Gain=2*wc_roll
  Gain2 : Gain  Gain=wc_roll^2
  Gain3 : Gain  Gain=-1
  Gain4 : Gain  Gain=-1
  Sum : Sum  Inputs=|++
  Sum1 : Sum  Inputs=|++
  Sum2 : Sum  Inputs=|+++
  U2 : Outport
  wires:
  ref_dot/1 -> Sum1/1
  x_hat/1 -> Bus Selector/1
  Bus Selector/3 -> Gain/1  "<x3>"
  Gain2/1 -> Sum2/1
  Gain/1 -> Sum2/3
  Gain1/1 -> Sum2/2
  Bus Selector/1 -> Gain4/1  "<x1>"
  Bus Selector/2 -> Gain3/1  "<x2>"
  Gain4/1 -> Sum/2
  Gain3/1 -> Sum1/2
  Sum1/1 -> Gain1/1
  Divide/1 -> U2/1
  ref/1 -> Sum/1
  Sum/1 -> Gain2/1
  Sum2/1 -> Divide/1
  Constant/1 -> Divide/2

== system testing/ADRC_roll/LESO1 ==
  phi : Inport
  U2 : Inport  Port=2
  Bus Creator : BusCreator  Inputs=3
  Gain : Gain  Gain=-beta1_roll
  Gain1 : Gain  Gain=-1
  Gain2 : Gain  Gain=-beta2_roll
  Gain3 : Gain  Gain=-beta3_roll
  Gain4 : Gain  Gain=b0_roll
  Integrator : Integrator
  Integrator1 : Integrator
  Integrator2 : Integrator
  Sum : Sum  Inputs=|++
  Sum1 : Sum  Inputs=|++
  Sum2 : Sum  Inputs=|+++
  z_hat : Outport
  wires:
  Gain4/1 -> Sum2/3
  U2/1 -> Gain4/1
  Sum2/1 -> Integrator1/1  "x2_dot"
  Gain2/1 -> Sum2/1
  Integrator2/1 -> Sum2/2, Bus Creator/3  "x3"
  Integrator1/1 -> Sum1/2, Bus Creator/2  "x2"
  Gain/1 -> Sum1/1
  Sum1/1 -> Integrator/1  "x1_dot"
  Bus Creator/1 -> z_hat/1
  Gain3/1 -> Integrator2/1  "x3_dot"
  Integrator/1 -> Sum/2, Bus Creator/1  "x1"
  Sum/1 -> Gain/1, Gain2/1, Gain3/1
  Gain1/1 -> Sum/1
  phi/1 -> Gain1/1

== system testing/ADRC_roll/TD1 ==
  v : Inport
  Constant11 : Constant  Value=r0_angle
  Constant12 : Constant  Value=h0
  Delay One Step : Delay  DelayLength=1  SampleTime=Ts
  Delay One Step1 : Delay  DelayLength=1  SampleTime=Ts
  Gain3 : Gain  Gain=Ts
  Gain4 : Gain  Gain=Ts
  Sum1 : Sum  Inputs=|++
  Sum6 : Sum  Inputs=|++
  Sum7 : Sum  Inputs=|+-
  fhan : MATLAB Function  TreatAsAtomicUnit=on
  ref : Outport
  dref : Outport  Port=2
  wires:
  v/1 -> Sum7/2
  Gain3/1 -> Sum6/1
  Constant12/1 -> fhan/4(h0)
  Delay One Step/1 -> Sum1/1
  Gain4/1 -> Sum1/2
  Sum1/1 -> Sum7/1, Delay One Step/1, ref/1  "v1"
  Sum7/1 -> fhan/1(e)
  fhan/1(u) -> Gain3/1
  Sum6/1 -> Delay One Step1/1  "v2"
  Constant11/1 -> fhan/3(r0)
  Delay One Step1/1 -> Gain4/1, Sum6/2, fhan/2(v2), dref/1

== system testing/ADRC_x/LADRC1 ==
  ref : Inport
  x_hat : Inport  Port=2
  ref_dot : Inport  Port=3
  Bus Selector : BusSelector  OutputSignals=x1,x2,x3
  Constant : Constant  Value=b0_x
  Divide : Product  Inputs=*/
  Gain : Gain  Gain=-1
  Gain1 : Gain  Gain=2*wc_x
  Gain2 : Gain  Gain=wc_x^2
  Gain3 : Gain  Gain=-1
  Gain4 : Gain  Gain=-1
  Sum : Sum  Inputs=|++
  Sum1 : Sum  Inputs=|++
  Sum2 : Sum  Inputs=|+++
  U1 : Outport
  wires:
  ref_dot/1 -> Sum1/1
  Divide/1 -> U1/1
  x_hat/1 -> Bus Selector/1
  Bus Selector/3 -> Gain/1  "<x3>"
  Gain2/1 -> Sum2/1
  Gain/1 -> Sum2/3
  Gain1/1 -> Sum2/2
  Bus Selector/1 -> Gain4/1  "<x1>"
  Bus Selector/2 -> Gain3/1  "<x2>"
  Gain4/1 -> Sum/2
  Gain3/1 -> Sum1/2
  Sum1/1 -> Gain1/1
  ref/1 -> Sum/1
  Sum/1 -> Gain2/1
  Sum2/1 -> Divide/1
  Constant/1 -> Divide/2

== system testing/ADRC_x/LESO1 ==
  x : Inport
  U1 : Inport  Port=2
  Bus Creator : BusCreator  Inputs=3
  Gain : Gain  Gain=-beta1_x
  Gain1 : Gain  Gain=-1
  Gain2 : Gain  Gain=-beta2_x
  Gain3 : Gain  Gain=-beta3_x
  Gain4 : Gain  Gain=b0_x
  Integrator : Integrator
  Integrator1 : Integrator
  Integrator2 : Integrator
  Sum : Sum  Inputs=|++
  Sum1 : Sum  Inputs=|++
  Sum2 : Sum  Inputs=|+++
  z_hat : Outport
  wires:
  Gain4/1 -> Sum2/3
  U1/1 -> Gain4/1
  Sum2/1 -> Integrator1/1  "x2_dot"
  Gain2/1 -> Sum2/1
  Integrator2/1 -> Sum2/2, Bus Creator/3  "x3"
  Integrator1/1 -> Sum1/2, Bus Creator/2  "x2"
  Gain/1 -> Sum1/1
  Sum1/1 -> Integrator/1  "x1_dot"
  Bus Creator/1 -> z_hat/1
  Gain3/1 -> Integrator2/1  "x3_dot"
  Integrator/1 -> Sum/2, Bus Creator/1  "x1"
  Sum/1 -> Gain/1, Gain2/1, Gain3/1
  Gain1/1 -> Sum/1
  x/1 -> Gain1/1

== system testing/ADRC_x/TD1 ==
  v : Inport
  Constant11 : Constant  Value=r0_position
  Constant12 : Constant  Value=h0
  Delay One Step : Delay  DelayLength=1  SampleTime=Ts
  Delay One Step1 : Delay  DelayLength=1  SampleTime=Ts
  Gain3 : Gain  Gain=Ts
  Gain4 : Gain  Gain=Ts
  Sum1 : Sum  Inputs=|++
  Sum6 : Sum  Inputs=|++
  Sum7 : Sum  Inputs=|+-
  fhan : MATLAB Function  TreatAsAtomicUnit=on
  ref : Outport
  dref : Outport  Port=2
  wires:
  v/1 -> Sum7/2
  Constant12/1 -> fhan/4(h0)
  Sum7/1 -> fhan/1(e)
  fhan/1(u) -> Gain3/1
  Constant11/1 -> fhan/3(r0)
  Delay One Step1/1 -> dref/1, fhan/2(v2), Sum6/2, Gain4/1
  Gain4/1 -> Sum1/2
  Sum1/1 -> ref/1, Sum7/1, Delay One Step/1  "v1"
  Sum6/1 -> Delay One Step1/1  "v2"
  Gain3/1 -> Sum6/1
  Delay One Step/1 -> Sum1/1

== system testing/ADRC_y/LADRC1 ==
  ref : Inport
  y_hat : Inport  Port=2
  ref_dot : Inport  Port=3
  Bus Selector : BusSelector  OutputSignals=x1,x2,x3
  Constant : Constant  Value=b0_y
  Divide : Product  Inputs=*/
  Gain : Gain  Gain=-1
  Gain1 : Gain  Gain=2*wc_y
  Gain2 : Gain  Gain=wc_y^2
  Gain3 : Gain  Gain=-1
  Gain4 : Gain  Gain=-1
  Sum : Sum  Inputs=|++
  Sum1 : Sum  Inputs=|++
  Sum2 : Sum  Inputs=|+++
  U1 : Outport
  wires:
  Sum/1 -> Gain2/1
  ref/1 -> Sum/1
  Sum1/1 -> Gain1/1
  Gain3/1 -> Sum1/2
  Gain4/1 -> Sum/2
  Bus Selector/2 -> Gain3/1  "<x2>"
  Bus Selector/1 -> Gain4/1  "<x1>"
  Gain1/1 -> Sum2/2
  Gain/1 -> Sum2/3
  Gain2/1 -> Sum2/1
  Bus Selector/3 -> Gain/1  "<x3>"
  y_hat/1 -> Bus Selector/1
  Divide/1 -> U1/1
  ref_dot/1 -> Sum1/1
  Sum2/1 -> Divide/1
  Constant/1 -> Divide/2

== system testing/ADRC_y/LESO1 ==
  y : Inport
  U1 : Inport  Port=2
  Bus Creator : BusCreator  Inputs=3
  Gain : Gain  Gain=-beta1_y
  Gain1 : Gain  Gain=-1
  Gain2 : Gain  Gain=-beta2_y
  Gain3 : Gain  Gain=-beta3_y
  Gain4 : Gain  Gain=b0_y
  Integrator : Integrator
  Integrator1 : Integrator
  Integrator2 : Integrator
  Sum : Sum  Inputs=|++
  Sum1 : Sum  Inputs=|++
  Sum2 : Sum  Inputs=|+++
  y_hat : Outport
  wires:
  y/1 -> Gain1/1
  Gain1/1 -> Sum/1
  Sum/1 -> Gain3/1, Gain2/1, Gain/1
  Integrator/1 -> Bus Creator/1, Sum/2  "x1"
  Gain3/1 -> Integrator2/1  "x3_dot"
  Bus Creator/1 -> y_hat/1
  Sum1/1 -> Integrator/1  "x1_dot"
  Gain/1 -> Sum1/1
  Integrator1/1 -> Bus Creator/2, Sum1/2  "x2"
  Integrator2/1 -> Bus Creator/3, Sum2/2  "x3"
  Gain2/1 -> Sum2/1
  Sum2/1 -> Integrator1/1  "x2_dot"
  U1/1 -> Gain4/1
  Gain4/1 -> Sum2/3

== system testing/ADRC_y/TD1 ==
  v : Inport
  Constant11 : Constant  Value=r0_position
  Constant12 : Constant  Value=h0
  Delay One Step : Delay  DelayLength=1  SampleTime=Ts
  Delay One Step1 : Delay  DelayLength=1  SampleTime=Ts
  Gain3 : Gain  Gain=Ts
  Gain4 : Gain  Gain=Ts
  Sum1 : Sum  Inputs=|++
  Sum6 : Sum  Inputs=|++
  Sum7 : Sum  Inputs=|+-
  fhan : MATLAB Function  TreatAsAtomicUnit=on
  ref : Outport
  dref : Outport  Port=2
  wires:
  v/1 -> Sum7/2
  Constant12/1 -> fhan/4(h0)
  Sum7/1 -> fhan/1(e)
  fhan/1(u) -> Gain3/1
  Constant11/1 -> fhan/3(r0)
  Delay One Step1/1 -> dref/1, fhan/2(v2), Sum6/2, Gain4/1
  Gain4/1 -> Sum1/2
  Sum1/1 -> ref/1, Sum7/1, Delay One Step/1  "v1"
  Sum6/1 -> Delay One Step1/1  "v2"
  Gain3/1 -> Sum6/1
  Delay One Step/1 -> Sum1/1

== system testing/ADRC_yaw/LADRC1 ==
  ref : Inport
  x_hat : Inport  Port=2
  ref_dot : Inport  Port=3
  Bus Selector : BusSelector  OutputSignals=x1,x2,x3
  Constant : Constant  Value=b0_yaw
  Divide : Product  Inputs=*/
  Gain : Gain  Gain=-1
  Gain1 : Gain  Gain=2*wc_yaw
  Gain2 : Gain  Gain=wc_yaw^2
  Gain3 : Gain  Gain=-1
  Gain4 : Gain  Gain=-1
  Sum : Sum  Inputs=|++
  Sum1 : Sum  Inputs=|++
  Sum2 : Sum  Inputs=|+++
  U1 : Outport
  wires:
  Sum/1 -> Gain2/1
  ref/1 -> Sum/1
  Sum1/1 -> Gain1/1
  Gain3/1 -> Sum1/2
  Gain4/1 -> Sum/2
  Bus Selector/2 -> Gain3/1  "<x2>"
  Bus Selector/1 -> Gain4/1  "<x1>"
  Gain1/1 -> Sum2/2
  Gain/1 -> Sum2/3
  Gain2/1 -> Sum2/1
  Bus Selector/3 -> Gain/1  "<x3>"
  x_hat/1 -> Bus Selector/1
  Divide/1 -> U1/1
  ref_dot/1 -> Sum1/1
  Sum2/1 -> Divide/1
  Constant/1 -> Divide/2

== system testing/ADRC_yaw/LESO1 ==
  theta : Inport
  U1 : Inport  Port=2
  Bus Creator : BusCreator  Inputs=3
  Gain : Gain  Gain=-beta1_yaw
  Gain1 : Gain  Gain=-1
  Gain2 : Gain  Gain=-beta2_yaw
  Gain3 : Gain  Gain=-beta3_yaw
  Gain4 : Gain  Gain=b0_yaw
  Integrator : Integrator
  Integrator1 : Integrator
  Integrator2 : Integrator
  Sum : Sum  Inputs=|++
  Sum1 : Sum  Inputs=|++
  Sum2 : Sum  Inputs=|+++
  z_hat : Outport
  wires:
  theta/1 -> Gain1/1
  Gain1/1 -> Sum/1
  Sum/1 -> Gain3/1, Gain2/1, Gain/1
  Integrator/1 -> Bus Creator/1, Sum/2  "x1"
  Gain3/1 -> Integrator2/1  "x3_dot"
  Bus Creator/1 -> z_hat/1
  Sum1/1 -> Integrator/1  "x1_dot"
  Gain/1 -> Sum1/1
  Integrator1/1 -> Bus Creator/2, Sum1/2  "x2"
  Integrator2/1 -> Bus Creator/3, Sum2/2  "x3"
  Gain2/1 -> Sum2/1
  Sum2/1 -> Integrator1/1  "x2_dot"
  U1/1 -> Gain4/1
  Gain4/1 -> Sum2/3

== system testing/ADRC_yaw/TD1 ==
  v : Inport
  Constant11 : Constant  Value=r0_angle
  Constant12 : Constant  Value=h0
  Delay One Step : Delay  DelayLength=1  SampleTime=Ts
  Delay One Step1 : Delay  DelayLength=1  SampleTime=Ts
  Gain3 : Gain  Gain=Ts
  Gain4 : Gain  Gain=Ts
  Sum1 : Sum  Inputs=|++
  Sum6 : Sum  Inputs=|++
  Sum7 : Sum  Inputs=|+-
  fhan : MATLAB Function  TreatAsAtomicUnit=on
  ref : Outport
  dref : Outport  Port=2
  wires:
  v/1 -> Sum7/2
  Gain3/1 -> Sum6/1
  Constant12/1 -> fhan/4(h0)
  Delay One Step/1 -> Sum1/1
  Gain4/1 -> Sum1/2
  Sum1/1 -> Sum7/1, Delay One Step/1, ref/1  "v1"
  Sum7/1 -> fhan/1(e)
  fhan/1(u) -> Gain3/1
  Sum6/1 -> Delay One Step1/1  "v2"
  Constant11/1 -> fhan/3(r0)
  Delay One Step1/1 -> Gain4/1, Sum6/2, fhan/2(v2), dref/1

== system testing/ADRC_z/LADRC1 ==
  ref : Inport
  x_hat : Inport  Port=2
  ref_dot : Inport  Port=3
  Bus Selector : BusSelector  OutputSignals=x1,x2,x3
  Constant1 : Constant  Value=b0_z
  Divide : Product  Inputs=*/
  Gain : Gain  Gain=-1
  Gain1 : Gain  Gain=2*wc_z
  Gain2 : Gain  Gain=wc_z^2
  Gain3 : Gain  Gain=-1
  Gain4 : Gain  Gain=-1
  Sum : Sum  Inputs=|++
  Sum1 : Sum  Inputs=|++
  Sum2 : Sum  Inputs=|+++
  U1 : Outport
  wires:
  ref_dot/1 -> Sum1/1
  Sum2/1 -> Divide/1
  x_hat/1 -> Bus Selector/1
  Bus Selector/3 -> Gain/1  "<x3>"
  Gain2/1 -> Sum2/1
  Gain/1 -> Sum2/3
  Gain1/1 -> Sum2/2
  Bus Selector/1 -> Gain4/1  "<x1>"
  Bus Selector/2 -> Gain3/1  "<x2>"
  Gain4/1 -> Sum/2
  Gain3/1 -> Sum1/2
  Sum1/1 -> Gain1/1
  Divide/1 -> U1/1
  Constant1/1 -> Divide/2
  ref/1 -> Sum/1
  Sum/1 -> Gain2/1

== system testing/ADRC_z/LESO1 ==
  z : Inport
  U1 : Inport  Port=2
  Bus Creator : BusCreator  Inputs=3
  Gain : Gain  Gain=-beta1_z
  Gain1 : Gain  Gain=-1
  Gain2 : Gain  Gain=-beta2_z
  Gain3 : Gain  Gain=-beta3_z
  Gain4 : Gain  Gain=b0_z
  Integrator : Integrator
  Integrator1 : Integrator
  Integrator2 : Integrator
  Sum : Sum  Inputs=|++
  Sum1 : Sum  Inputs=|++
  Sum2 : Sum  Inputs=|+++
  z_hat : Outport
  wires:
  Gain4/1 -> Sum2/3
  U1/1 -> Gain4/1
  Sum2/1 -> Integrator1/1  "x2_dot"
  Gain2/1 -> Sum2/1
  Integrator2/1 -> Sum2/2, Bus Creator/3  "x3"
  Integrator1/1 -> Sum1/2, Bus Creator/2  "x2"
  Gain/1 -> Sum1/1
  Sum1/1 -> Integrator/1  "x1_dot"
  Bus Creator/1 -> z_hat/1
  Gain3/1 -> Integrator2/1  "x3_dot"
  Integrator/1 -> Sum/2, Bus Creator/1  "x1"
  Sum/1 -> Gain/1, Gain2/1, Gain3/1
  Gain1/1 -> Sum/1
  z/1 -> Gain1/1

== system testing/ADRC_z/TD1 ==
  v : Inport
  Constant11 : Constant  Value=r0_position
  Constant12 : Constant  Value=h0
  Delay One Step : Delay  DelayLength=1  SampleTime=Ts
  Delay One Step1 : Delay  DelayLength=1  SampleTime=Ts
  Gain3 : Gain  Gain=Ts
  Gain4 : Gain  Gain=Ts
  Sum1 : Sum  Inputs=|++
  Sum6 : Sum  Inputs=|++
  Sum7 : Sum  Inputs=|+-
  fhan : MATLAB Function  TreatAsAtomicUnit=on
  ref : Outport
  dref : Outport  Port=2
  wires:
  v/1 -> Sum7/2
  Constant12/1 -> fhan/4(h0)
  Sum7/1 -> fhan/1(e)
  fhan/1(u) -> Gain3/1
  Constant11/1 -> fhan/3(r0)
  Delay One Step1/1 -> dref/1, fhan/2(v2), Sum6/2, Gain4/1
  Gain4/1 -> Sum1/2
  Sum1/1 -> ref/1, Sum7/1, Delay One Step/1  "v1"
  Sum6/1 -> Delay One Step1/1  "v2"
  Gain3/1 -> Sum6/1
  Delay One Step/1 -> Sum1/1

== system testing/Force & Torque to Speeds/Speed to Force & Torque3 ==
  In1 : Inport
  Constant1 : Constant  Value=Alloc_2
  Matrix Multiply1 : Product  Multiplication=Matrix(*)
  U : Outport
  wires:
  Constant1/1 -> Matrix Multiply1/1
  Matrix Multiply1/1 -> U/1
  In1/1 -> Matrix Multiply1/2  "Omega^2"

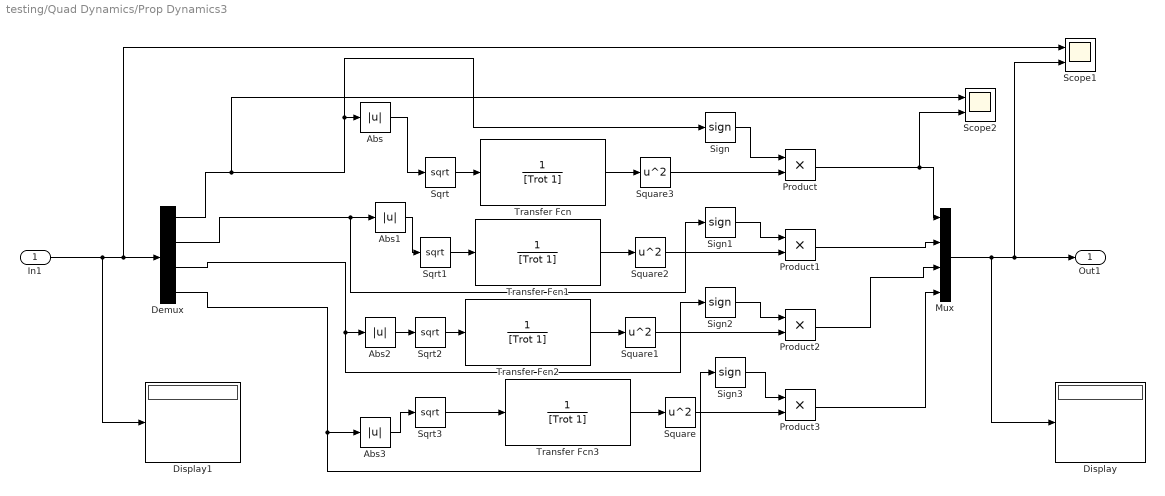
== system testing/Quad Dynamics/Prop Dynamics3 ==
  In1 : Inport
  Abs{,1..3} (4 alike) : Abs  SaturateOnIntegerOverflow=off
  Demux : Demux
  Display : Display
  Display1 : Display
  Mux : Mux
  Product{,1..3} (4 alike) : Product
  Scope1 : Scope  NumInputPorts=2
      settings: ActiveDisplayYMinimum=112181.7837613984  ActiveDisplayYMaximum=826252.36344831332  DataLoggingVariableName=ScopeData22
  Scope2 : Scope  NumInputPorts=2
      settings: ActiveDisplayYMinimum=474145.79333634069  ActiveDisplayYMaximum=566090.11578068486  DataLoggingVariableName=ScopeData26
  Sign{,1..3} (4 alike) : Signum
  Sqrt{,1..3} (4 alike) : Sqrt
  Square{,1..3} (4 alike) : Math  Operator=square
  Transfer Fcn{,1..3} (4 alike) : TransferFcn  Denominator=[Trot 1]
  Out1 : Outport
  wires:
  Sign3/1 -> Product3/1
  Sign2/1 -> Product2/1
  Sign1/1 -> Product1/1
  Sign/1 -> Product/1
  Product3/1 -> Mux/4
  Abs3/1 -> Sqrt3/1
  Abs2/1 -> Sqrt2/1
  Abs1/1 -> Sqrt1/1
  Abs/1 -> Sqrt/1
  Square3/1 -> Product/2
  Square2/1 -> Product1/2
  Square1/1 -> Product2/2
  Square/1 -> Product3/2
  Sqrt3/1 -> Transfer Fcn3/1
  Sqrt2/1 -> Transfer Fcn2/1
  Sqrt1/1 -> Transfer Fcn1/1
  Sqrt/1 -> Transfer Fcn/1
  Transfer Fcn3/1 -> Square/1
  Transfer Fcn2/1 -> Square1/1
  Transfer Fcn/1 -> Square3/1
  Transfer Fcn1/1 -> Square2/1
  Mux/1 -> Scope1/2, Out1/1, Display/1
  In1/1 -> Scope1/1, Demux/1, Display1/1
  Demux/1 -> Scope2/1, Abs/1, Sign/1
  Demux/2 -> Sign1/1, Abs1/1
  Demux/3 -> Abs2/1, Sign2/1
  Demux/4 -> Abs3/1, Sign3/1
  Product/1 -> Scope2/2, Mux/1
  Product1/1 -> Mux/2
  Product2/1 -> Mux/3

== system testing/Quad Dynamics/Speed to Force & Torque3 ==
  In1 : Inport
  Constant1 : Constant  Value=Alloc_2
  Matrix Multiply1 : Product  Multiplication=Matrix(*)
  U : Outport
  wires:
  Constant1/1 -> Matrix Multiply1/1
  Matrix Multiply1/1 -> U/1
  In1/1 -> Matrix Multiply1/2  "Omega^2"
